simulink model "AFC_FFNN_trainlm_15_15_15_NoSat_Jan_23_RepFast"  (R2021a)
settings: Solver=ode15s  StartTime=0.0  StopTime=T  MaxStep=.01  RelTol=1e-3
undefined symbols (not defined in the file): AF_sensor_tol, fault_time, fuel_inj_tol, kappa_tol, MAF_sensor_tol, patch_sig, pump_tol, safe_patch_sig, sw, tau_ww_tol
libraries: neural x50, simulink x3
(part 2 of 2)

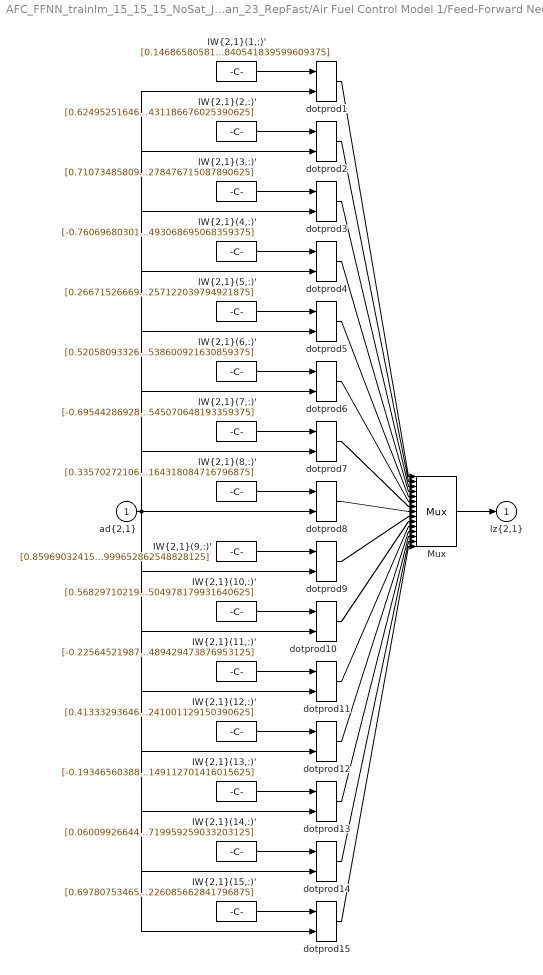
== system AFC_FFNN_trainlm_15_15_15_NoSat_Jan_23_RepFast/Air Fuel Control Model 1/Feed-Forward Neural Network/Layer 2/LW{2,1} ==
  "ad{2,1}" : Inport  PortDimensions=15
      mask Display: e = 0.06;c1 = [120 230 180]/255;c2 = ([120 230 180]+0)/(256+128);c3 = ([120 230 180]+128)/(256+128);patch([0 1 1 0],[0 0 1 1],c1);patch([0 1 1 1-e 1-e 0+e],[0 0 1 1-e 0+e 0+e],c2);patch([0 0 1 1-e 0+e 0+e],[0 1 1 1-e 1-e 0+e],c3);plot([0 1 1 0 0],[0 0 1 1 0]);
  "IW{2,1}(1,:)'" : Constant  Value=[0.1468658058110374753368887468241155147552490234375;-0.79986890826566170442646352967130951583385467529296875;-0.31412633700742986775367171503603458404541015625;-0.00332579596645567361623552216087773558683693408966064453125;0.1312237814313217398876076913438737392425537109375;0.344524720263148787058327116028522141277790069580078125;-0.0408263490105180704148324366542510688304901123046875;-0.197143189425145581861187338290619663894176483154296875;-0.211467920088183103377588167859357781708240509033203125;-0.0228887593846358594618095594341866672039031982421875;0.9727483047205953692326829695957712829113006591796875;-0.15275385755570081158793982467614114284515380859375;0.448998803742126473270701580986496992409229278564453125;0.1435643437851705783714351127855479717254638671875;0.9935339892538654904541317591792903840541839599609375]
      mask Display: e = 0.06;c1 = [120 150 230]/255;c2 = ([120 150 230]+0)/383;c3 = ([120 150 230]+128)/383;patch([0 1 1 0],[0 0 1 1],c1);patch([0 1 1 1-e 1-e 0+e],[0 0 1 1-e 0+e 0+e],c2);patch([0 0 1 1-e 0+e 0+e],[0 1 1 1-e 1-e 0+e],c3);plot([0 1 1 0 0],[0 0 1 1 0]);disp('weights');
  "IW{2,1}(10,:)'" : Constant  Value=[0.5682971021935003808067676800419576466083526611328125;-0.7275100622197581134997790286433883011341094970703125;1.4406360212981699220335940481163561344146728515625;-0.7098343326217027016156180252437479794025421142578125;0.3745290668992009575077872796100564301013946533203125;-0.0614067373898913027030488365198834799230098724365234375;0.964924509608335423394009922049008309841156005859375;-1.3273865141156055980076189371175132691860198974609375;-0.203156115681673465900303199305199086666107177734375;-0.7408998901019552274505031164153479039669036865234375;1.0233270938010277095742139863432385027408599853515625;0.69404582667213154945073938506538979709148406982421875;-0.23685294970424097815708819325664080679416656494140625;-0.0126849048783663764794482631259597837924957275390625;-0.244330775780726927592922947951592504978179931640625]
      mask Display: e = 0.06;c1 = [120 150 230]/255;c2 = ([120 150 230]+0)/383;c3 = ([120 150 230]+128)/383;patch([0 1 1 0],[0 0 1 1],c1);patch([0 1 1 1-e 1-e 0+e],[0 0 1 1-e 0+e 0+e],c2);patch([0 0 1 1-e 0+e 0+e],[0 1 1 1-e 1-e 0+e],c3);plot([0 1 1 0 0],[0 0 1 1 0]);disp('weights');
  "IW{2,1}(11,:)'" : Constant  Value=[-0.2256452198759715255249602705589495599269866943359375;0.727956654138967262923642920213751494884490966796875;-0.5453793247586904424650811051833443343639373779296875;0.547967139390781898811155770090408623218536376953125;-0.1828759723086506028266740031540393829345703125;0.9374135951140996070307664922438561916351318359375;0.87270401334910641111264339997433125972747802734375;0.853037029850580719170238808146677911281585693359375;0.1825800053059129790522518987927469424903392791748046875;-0.7678337019231407101216291266609914600849151611328125;0.421204976982361978254942869170918129384517669677734375;-0.0579419915609621638541426591473282314836978912353515625;0.5795506990507470757023611440672539174556732177734375;-0.477128967133783277176917181350290775299072265625;-0.670782654299447944623580042389221489429473876953125]
      mask Display: e = 0.06;c1 = [120 150 230]/255;c2 = ([120 150 230]+0)/383;c3 = ([120 150 230]+128)/383;patch([0 1 1 0],[0 0 1 1],c1);patch([0 1 1 1-e 1-e 0+e],[0 0 1 1-e 0+e 0+e],c2);patch([0 0 1 1-e 0+e 0+e],[0 1 1 1-e 1-e 0+e],c3);plot([0 1 1 0 0],[0 0 1 1 0]);disp('weights');
  "IW{2,1}(12,:)'" : Constant  Value=[0.41333293646864799342210972099564969539642333984375;-0.8616022116206336622923345203162170946598052978515625;-0.348616050190197535041392029597773216664791107177734375;-0.5692780055831174745861744668218307197093963623046875;0.9529144783762959480810650347848422825336456298828125;-1.0241829268729427671047460535191930830478668212890625;0.5831636473464032466296202983357943594455718994140625;0.499306613814386957006519196511362679302692413330078125;0.6451270201528844783211980029591359198093414306640625;0.2605675373402061012484409729950129985809326171875;-0.01491909072521746537631770479492843151092529296875;-0.167342895014342241122307086698128841817378997802734375;-0.562609182407641572609691138495691120624542236328125;-0.2562071576988582677358863293193280696868896484375;-0.3877593402600434391302997028105892241001129150390625]
      mask Display: e = 0.06;c1 = [120 150 230]/255;c2 = ([120 150 230]+0)/383;c3 = ([120 150 230]+128)/383;patch([0 1 1 0],[0 0 1 1],c1);patch([0 1 1 1-e 1-e 0+e],[0 0 1 1-e 0+e 0+e],c2);patch([0 0 1 1-e 0+e 0+e],[0 1 1 1-e 1-e 0+e],c3);plot([0 1 1 0 0],[0 0 1 1 0]);disp('weights');
  "IW{2,1}(13,:)'" : Constant  Value=[-0.1934656038895019580792222768650390207767486572265625;-0.2390404906948966068380713068108889274299144744873046875;-0.1199124406723394986595820910224574618041515350341796875;0.263449521186924773274995459360070526599884033203125;0.4440977442440028344350366751314140856266021728515625;0.53872301524054255761342346886522136628627777099609375;-0.2115765017478363763103743622195906937122344970703125;-0.6234500873564188250242068534134887158870697021484375;-0.35608968297847898298869040445424616336822509765625;-0.49677879715403161497988548944704234600067138671875;0.419241740090347481118016048640129156410694122314453125;-0.33564242304183000698003525030799210071563720703125;0.433229749317704027067321703725610859692096710205078125;0.460056404944834351766758118174038827419281005859375;-0.256260589179901021594787380308844149112701416015625]
      mask Display: e = 0.06;c1 = [120 150 230]/255;c2 = ([120 150 230]+0)/383;c3 = ([120 150 230]+128)/383;patch([0 1 1 0],[0 0 1 1],c1);patch([0 1 1 1-e 1-e 0+e],[0 0 1 1-e 0+e 0+e],c2);patch([0 0 1 1-e 0+e 0+e],[0 1 1 1-e 1-e 0+e],c3);plot([0 1 1 0 0],[0 0 1 1 0]);disp('weights');
  "IW{2,1}(14,:)'" : Constant  Value=[0.0600992664475967774961873146821744740009307861328125;-0.65050183753509538409076640164130367338657379150390625;1.362085994538364541739383639651350677013397216796875;0.042474272203300279804327743704561726190149784088134765625;-0.2568578517627091439834430275368504226207733154296875;0.81744135101609993743210225147777236998081207275390625;-0.2498833666170330314315606301533989608287811279296875;-0.10525015327370969286935320496922940947115421295166015625;0.03216246871763693560009045313563547097146511077880859375;-0.502647721643322942242093631648458540439605712890625;-0.3867159297211497648305567054194398224353790283203125;0.73794130222845388811236944093252532184123992919921875;0.023130893299841949473094615541413077153265476226806640625;0.1348448958576984324508885038085281848907470703125;-0.3121945271696671131422817779821343719959259033203125]
      mask Display: e = 0.06;c1 = [120 150 230]/255;c2 = ([120 150 230]+0)/383;c3 = ([120 150 230]+128)/383;patch([0 1 1 0],[0 0 1 1],c1);patch([0 1 1 1-e 1-e 0+e],[0 0 1 1-e 0+e 0+e],c2);patch([0 0 1 1-e 0+e 0+e],[0 1 1 1-e 1-e 0+e],c3);plot([0 1 1 0 0],[0 0 1 1 0]);disp('weights');
  "IW{2,1}(15,:)'" : Constant  Value=[0.6978075346578351823012553722946904599666595458984375;-0.73662106818013228792807467470993287861347198486328125;-1.1123650153279764918323735400917939841747283935546875;-0.11030835599876363806171042369896895252168178558349609375;0.734200051032391609595606496441178023815155029296875;-0.1876468311379226872048775476287119090557098388671875;0.7184828013258843792954166929121129214763641357421875;0.60013058592138601721188706505927257239818572998046875;0.053448907742239711027298909584715147502720355987548828125;0.9120261675330609829615013950387947261333465576171875;0.74302316527727463313368616582010872662067413330078125;-0.4149924922329122356501329704769887030124664306640625;0.8172177093320953655819494088063947856426239013671875;0.9305593583416114089601478553959168493747711181640625;-0.06823078255388548285509386914782226085662841796875]
      mask Display: e = 0.06;c1 = [120 150 230]/255;c2 = ([120 150 230]+0)/383;c3 = ([120 150 230]+128)/383;patch([0 1 1 0],[0 0 1 1],c1);patch([0 1 1 1-e 1-e 0+e],[0 0 1 1-e 0+e 0+e],c2);patch([0 0 1 1-e 0+e 0+e],[0 1 1 1-e 1-e 0+e],c3);plot([0 1 1 0 0],[0 0 1 1 0]);disp('weights');
  "IW{2,1}(2,:)'" : Constant  Value=[0.6249525164608675797950354535714723169803619384765625;0.412890681297754802425714615310425870120525360107421875;-0.2159788554806470750602187536060228012502193450927734375;0.3508923949942845954552694820449687540531158447265625;-0.1422183036643251963226930456585250794887542724609375;0.612312898614546075037878836155869066715240478515625;-0.48507316554088220073026604950428009033203125;-0.64878999441310247764391760938451625406742095947265625;-0.7391660575102572128258771044784225523471832275390625;-0.086116803229575378253457529353909194469451904296875;0.5698654964419118673646380557329393923282623291015625;0.7165517327928829782734965192503295838832855224609375;-0.464988407736367237443886324399500153958797454833984375;-0.6335294236047517291154917984385974705219268798828125;-0.0748668890844010892493542996817268431186676025390625]
      mask Display: e = 0.06;c1 = [120 150 230]/255;c2 = ([120 150 230]+0)/383;c3 = ([120 150 230]+128)/383;patch([0 1 1 0],[0 0 1 1],c1);patch([0 1 1 1-e 1-e 0+e],[0 0 1 1-e 0+e 0+e],c2);patch([0 0 1 1-e 0+e 0+e],[0 1 1 1-e 1-e 0+e],c3);plot([0 1 1 0 0],[0 0 1 1 0]);disp('weights');
  "IW{2,1}(3,:)'" : Constant  Value=[0.7107348580942822735551089863292872905731201171875;-0.342239153986161337428484330303035676479339599609375;-0.19023870928318320494554427568800747394561767578125;-0.8599175367517801760186557658016681671142578125;0.32990234960410713682676941971294581890106201171875;0.000120624052140971826929671806283295154571533203125;-0.5464970238293351822989052379853092133998870849609375;0.4014662532458366239751512694056145846843719482421875;0.2334039403776750898344971574260853230953216552734375;0.039564090317298905574716627597808837890625;-0.425583977343654940028727651224471628665924072265625;0.79559741585239596162182351690717041492462158203125;-0.183333770828677966591158110531978309154510498046875;-0.665380052920768516599991926341317594051361083984375;-0.09104362918916653057976873242296278476715087890625]
      mask Display: e = 0.06;c1 = [120 150 230]/255;c2 = ([120 150 230]+0)/383;c3 = ([120 150 230]+128)/383;patch([0 1 1 0],[0 0 1 1],c1);patch([0 1 1 1-e 1-e 0+e],[0 0 1 1-e 0+e 0+e],c2);patch([0 0 1 1-e 0+e 0+e],[0 1 1 1-e 1-e 0+e],c3);plot([0 1 1 0 0],[0 0 1 1 0]);disp('weights');
  "IW{2,1}(4,:)'" : Constant  Value=[-0.7606968030107481570922800528933294117450714111328125;-0.7535509674089102549743302006390877068042755126953125;-0.0455651968607446722359100022003985941410064697265625;-0.4725010400413507394290490992716513574123382568359375;0.7174803353217551471487922754022292792797088623046875;-0.3329299845408628666376671390025876462459564208984375;0.6842857552629875161898098667734302580356597900390625;-0.4818920562347488445453791428008116781711578369140625;0.8353636929366297092514059841050766408443450927734375;0.3770512178109644008117129487800411880016326904296875;0.7827280064979384999190870075835846364498138427734375;0.6009678795926596261978147595073096454143524169921875;-0.226909272979972431727446746663190424442291259765625;0.4638849660490063087081580306403338909149169921875;-0.6100135079769015700179579653195105493068695068359375]
      mask Display: e = 0.06;c1 = [120 150 230]/255;c2 = ([120 150 230]+0)/383;c3 = ([120 150 230]+128)/383;patch([0 1 1 0],[0 0 1 1],c1);patch([0 1 1 1-e 1-e 0+e],[0 0 1 1-e 0+e 0+e],c2);patch([0 0 1 1-e 0+e 0+e],[0 1 1 1-e 1-e 0+e],c3);plot([0 1 1 0 0],[0 0 1 1 0]);disp('weights');
  "IW{2,1}(5,:)'" : Constant  Value=[0.266715266696730513018565034144558012485504150390625;-0.332533963167412849326609602940152399241924285888671875;0.46985499617614345790883589870645664632320404052734375;-0.76651164888252265594559275996289215981960296630859375;-0.027119185528958755782014122814871370792388916015625;0.70201174892076012579167354488163255155086517333984375;-0.4255423106365061602929245054838247597217559814453125;-0.2801603963093963756136872689239680767059326171875;-1.091708492451566758774106347118504345417022705078125;-0.0635774578716965521607562550343573093414306640625;0.02153832134551721122495138160957139916718006134033203125;-0.5143365196906428682410705732763744890689849853515625;-0.67841812849830451792598751126206479966640472412109375;0.931788859196381213934046172653324902057647705078125;-0.0385504692749076838254040922038257122039794921875]
      mask Display: e = 0.06;c1 = [120 150 230]/255;c2 = ([120 150 230]+0)/383;c3 = ([120 150 230]+128)/383;patch([0 1 1 0],[0 0 1 1],c1);patch([0 1 1 1-e 1-e 0+e],[0 0 1 1-e 0+e 0+e],c2);patch([0 0 1 1-e 0+e 0+e],[0 1 1 1-e 1-e 0+e],c3);plot([0 1 1 0 0],[0 0 1 1 0]);disp('weights');
  "IW{2,1}(6,:)'" : Constant  Value=[0.5205809332657251875531301266164518892765045166015625;0.369459481161023450823677194421179592609405517578125;0.6135047231561936431631920640938915312290191650390625;0.059136244425769035615303437225520610809326171875;0.374148337822167054156352605787105858325958251953125;-0.9186599140957822928754694657982327044010162353515625;-0.599107887517563053592084543197415769100189208984375;-0.4882174416335660627197512440034188330173492431640625;-0.85474982889113704231931478716433048248291015625;-0.599702408658733698842979720211587846279144287109375;0.2338031628062349209784542836132459342479705810546875;0.4616289121641188319955517727066762745380401611328125;-0.3749002843746840341054848977364599704742431640625;-0.4338786459236596559918552884482778608798980712890625;0.885425136431036374773384522995911538600921630859375]
      mask Display: e = 0.06;c1 = [120 150 230]/255;c2 = ([120 150 230]+0)/383;c3 = ([120 150 230]+128)/383;patch([0 1 1 0],[0 0 1 1],c1);patch([0 1 1 1-e 1-e 0+e],[0 0 1 1-e 0+e 0+e],c2);patch([0 0 1 1-e 0+e 0+e],[0 1 1 1-e 1-e 0+e],c3);plot([0 1 1 0 0],[0 0 1 1 0]);disp('weights');
  "IW{2,1}(7,:)'" : Constant  Value=[-0.695442869286326814659560113796032965183258056640625;-0.881550976945969733122865363839082419872283935546875;0.8093922409587241961759218611405231058597564697265625;0.09552673732521850535892582456654054112732410430908203125;0.4068000332342711633515364155755378305912017822265625;0.37250243473358002344042461118078790605068206787109375;0.6941789590380762486887533668777905404567718505859375;0.63902927140569254493840389841352589428424835205078125;-0.396592890196696412630217309924773871898651123046875;-0.5169744106628451074669783338322304189205169677734375;-0.60043822969177307324883940964355133473873138427734375;0.55133135124757604028644664140301756560802459716796875;0.1855228100993589201994637960524414665997028350830078125;-0.7646540500302252407749392659752629697322845458984375;-0.5250407508751633312016338095418177545070648193359375]
      mask Display: e = 0.06;c1 = [120 150 230]/255;c2 = ([120 150 230]+0)/383;c3 = ([120 150 230]+128)/383;patch([0 1 1 0],[0 0 1 1],c1);patch([0 1 1 1-e 1-e 0+e],[0 0 1 1-e 0+e 0+e],c2);patch([0 0 1 1-e 0+e 0+e],[0 1 1 1-e 1-e 0+e],c3);plot([0 1 1 0 0],[0 0 1 1 0]);disp('weights');
  "IW{2,1}(8,:)'" : Constant  Value=[0.335702721066147180550842676893807947635650634765625;-0.6234135387209367440419782724347896873950958251953125;0.05600270005710324128234134377635200507938861846923828125;0.738664641377198449845309369266033172607421875;-0.8518457958148861752789571255561895668506622314453125;0.1699491832068246999210003878033603541553020477294921875;0.9024625642331134400819792062975466251373291015625;0.1858132442856689492405308783418149687349796295166015625;-0.83828507014463971014350818222737871110439300537109375;0.336524452681205676896070144721306860446929931640625;-0.62012758117489708009628657237044535577297210693359375;0.6610380858166651218965625957935117185115814208984375;-0.009806907065873525508603592015788308344781398773193359375;-0.012782031693472806210820635897107422351837158203125;0.2179003717440213261369308384018950164318084716796875]
      mask Display: e = 0.06;c1 = [120 150 230]/255;c2 = ([120 150 230]+0)/383;c3 = ([120 150 230]+128)/383;patch([0 1 1 0],[0 0 1 1],c1);patch([0 1 1 1-e 1-e 0+e],[0 0 1 1-e 0+e 0+e],c2);patch([0 0 1 1-e 0+e 0+e],[0 1 1 1-e 1-e 0+e],c3);plot([0 1 1 0 0],[0 0 1 1 0]);disp('weights');
  "IW{2,1}(9,:)'" : Constant  Value=[0.8596903241516711258185523547581396996974945068359375;0.5446400156727084773677916018641553819179534912109375;-8.868221093991540016077124164439737796783447265625;-0.63033703012778452556830188768799416720867156982421875;0.2101733469269653209465786858345381915569305419921875;0.6476803619839068826280481516732834279537200927734375;-0.884327548513141881159071999718435108661651611328125;0.45028320308204128341600380736053921282291412353515625;-0.61726588006551230680685193874523974955081939697265625;0.8963735042713738554454039331176318228244781494140625;-0.66039547280161359221750672077178023755550384521484375;-0.1518690387460164270549967113765887916088104248046875;-0.0875557235233536956808819695652346126735210418701171875;-0.32870025966817717488765993039123713970184326171875;-0.7543531819149951189729108591563999652862548828125]
      mask Display: e = 0.06;c1 = [120 150 230]/255;c2 = ([120 150 230]+0)/383;c3 = ([120 150 230]+128)/383;patch([0 1 1 0],[0 0 1 1],c1);patch([0 1 1 1-e 1-e 0+e],[0 0 1 1-e 0+e 0+e],c2);patch([0 0 1 1-e 0+e 0+e],[0 1 1 1-e 1-e 0+e],c3);plot([0 1 1 0 0],[0 0 1 1 0]);disp('weights');
  Mux : Mux  Inputs=15
      mask Display: e = 0.06;c1 = [120 150 230]/255;c2 = ([120 150 230]+0)/383;c3 = ([120 150 230]+128)/383;patch([0 1 1 0],[0 0 1 1],c1);patch([0 1 1 1-e 1-e 0+e],[0 0 1 1-e 0+e 0+e],c2);patch([0 0 1 1-e 0+e 0+e],[0 1 1 1-e 1-e 0+e],c3);plot([0 1 1 0 0],[0 0 1 1 0]);disp('Mux');
  dotprod{1..15} (15 alike) : neural/Weight Functions/dotprod
  "lz{2,1}" : Outport
      mask Display: e = 0.06;c1 = [120 230 180]/255;c2 = ([120 230 180]+0)/(256+128);c3 = ([120 230 180]+128)/(256+128);patch([0 1 1 0],[0 0 1 1],c1);patch([0 1 1 1-e 1-e 0+e],[0 0 1 1-e 0+e 0+e],c2);patch([0 0 1 1-e 0+e 0+e],[0 1 1 1-e 1-e 0+e],c3);plot([0 1 1 0 0],[0 0 1 1 0]);
  wires:
  "IW{2,1}(1,:)'"/1 -> dotprod1/1
  "ad{2,1}"/1 -> dotprod1/2, dotprod2/2, dotprod3/2, dotprod4/2, dotprod5/2, dotprod6/2, dotprod7/2, dotprod8/2, dotprod9/2, dotprod10/2, dotprod11/2, dotprod12/2, dotprod13/2, dotprod14/2, dotprod15/2
  dotprod1/1 -> Mux/1
  "IW{2,1}(2,:)'"/1 -> dotprod2/1
  dotprod2/1 -> Mux/2
  "IW{2,1}(3,:)'"/1 -> dotprod3/1
  dotprod3/1 -> Mux/3
  "IW{2,1}(4,:)'"/1 -> dotprod4/1
  dotprod4/1 -> Mux/4
  "IW{2,1}(5,:)'"/1 -> dotprod5/1
  dotprod5/1 -> Mux/5
  "IW{2,1}(6,:)'"/1 -> dotprod6/1
  dotprod6/1 -> Mux/6
  "IW{2,1}(7,:)'"/1 -> dotprod7/1
  dotprod7/1 -> Mux/7
  "IW{2,1}(8,:)'"/1 -> dotprod8/1
  dotprod8/1 -> Mux/8
  "IW{2,1}(9,:)'"/1 -> dotprod9/1
  dotprod9/1 -> Mux/9
  "IW{2,1}(10,:)'"/1 -> dotprod10/1
  dotprod10/1 -> Mux/10
  "IW{2,1}(11,:)'"/1 -> dotprod11/1
  dotprod11/1 -> Mux/11
  "IW{2,1}(12,:)'"/1 -> dotprod12/1
  dotprod12/1 -> Mux/12
  "IW{2,1}(13,:)'"/1 -> dotprod13/1
  dotprod13/1 -> Mux/13
  "IW{2,1}(14,:)'"/1 -> dotprod14/1
  dotprod14/1 -> Mux/14
  "IW{2,1}(15,:)'"/1 -> dotprod15/1
  dotprod15/1 -> Mux/15
  Mux/1 -> "lz{2,1}"/1

== system AFC_FFNN_trainlm_15_15_15_NoSat_Jan_23_RepFast/Air Fuel Control Model 1/Feed-Forward Neural Network/Layer 3/Delays 1 ==
  "p{3}" : Inport  PortDimensions=15
      mask Display: e = 0.06;c1 = [120 230 180]/255;c2 = ([120 230 180]+0)/(256+128);c3 = ([120 230 180]+128)/(256+128);patch([0 1 1 0],[0 0 1 1],c1);patch([0 1 1 1-e 1-e 0+e],[0 0 1 1-e 0+e 0+e],c2);patch([0 0 1 1-e 0+e 0+e],[0 1 1 1-e 1-e 0+e],c3);plot([0 1 1 0 0],[0 0 1 1 0]);
  mux : Mux  Inputs=1
      mask Display: e = 0.06;c1 = [120 150 230]/255;c2 = ([120 150 230]+0)/383;c3 = ([120 150 230]+128)/383;patch([0 1 1 0],[0 0 1 1],c1);patch([0 1 1 1-e 1-e 0+e],[0 0 1 1-e 0+e 0+e],c2);patch([0 0 1 1-e 0+e 0+e],[0 1 1 1-e 1-e 0+e],c3);plot([0 1 1 0 0],[0 0 1 1 0]);disp('Mux')
  "pd{3,2}" : Outport
      mask Display: e = 0.06;c1 = [120 230 180]/255;c2 = ([120 230 180]+0)/(256+128);c3 = ([120 230 180]+128)/(256+128);patch([0 1 1 0],[0 0 1 1],c1);patch([0 1 1 1-e 1-e 0+e],[0 0 1 1-e 0+e 0+e],c2);patch([0 0 1 1-e 0+e 0+e],[0 1 1 1-e 1-e 0+e],c3);plot([0 1 1 0 0],[0 0 1 1 0]);
  wires:
  "p{3}"/1 -> mux/1
  mux/1 -> "pd{3,2}"/1

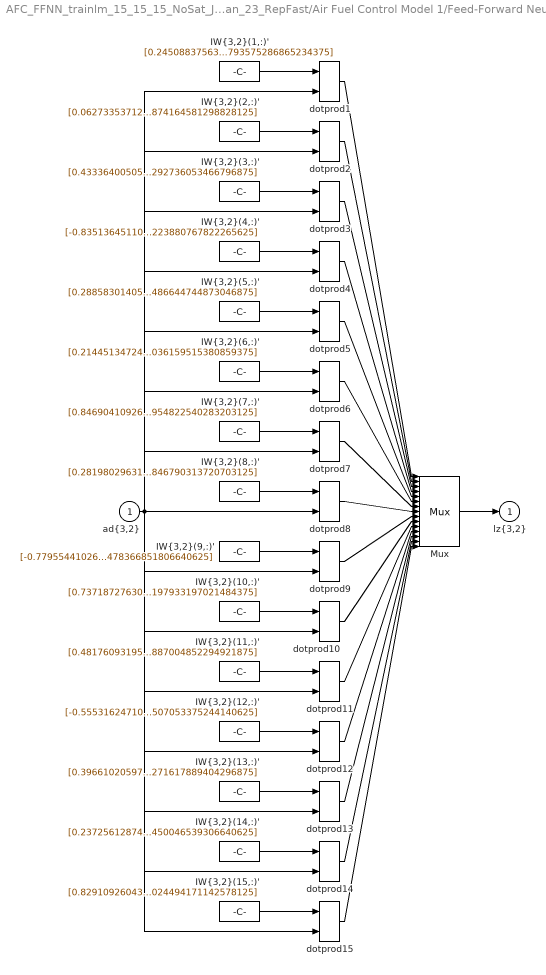
== system AFC_FFNN_trainlm_15_15_15_NoSat_Jan_23_RepFast/Air Fuel Control Model 1/Feed-Forward Neural Network/Layer 3/LW{3,2} ==
  "ad{3,2}" : Inport  PortDimensions=15
      mask Display: e = 0.06;c1 = [120 230 180]/255;c2 = ([120 230 180]+0)/(256+128);c3 = ([120 230 180]+128)/(256+128);patch([0 1 1 0],[0 0 1 1],c1);patch([0 1 1 1-e 1-e 0+e],[0 0 1 1-e 0+e 0+e],c2);patch([0 0 1 1-e 0+e 0+e],[0 1 1 1-e 1-e 0+e],c3);plot([0 1 1 0 0],[0 0 1 1 0]);
  "IW{3,2}(1,:)'" : Constant  Value=[0.245088375632908306300805634236894547939300537109375;-0.9630654315301534484916601286386139690876007080078125;0.9600091175752567540513382482458837330341339111328125;0.845118910397417710811396318604238331317901611328125;-0.7176582003307065971142719718045555055141448974609375;-0.589273318857662875558389714569784700870513916015625;-0.953421768699953542380853832582943141460418701171875;0.1957236320591506650856672422378323972225189208984375;0.1829565434390272304909785816562362015247344970703125;-0.7818743407298061054433446770417504012584686279296875;-0.93223551791788850096054375171661376953125;0.426672705339178559569290882791392505168914794921875;0.662323204252165620431469506002031266689300537109375;-0.25531274000819781377913386677391827106475830078125;0.3872106486699615768287685568793676793575286865234375]
      mask Display: e = 0.06;c1 = [120 150 230]/255;c2 = ([120 150 230]+0)/383;c3 = ([120 150 230]+128)/383;patch([0 1 1 0],[0 0 1 1],c1);patch([0 1 1 1-e 1-e 0+e],[0 0 1 1-e 0+e 0+e],c2);patch([0 0 1 1-e 0+e 0+e],[0 1 1 1-e 1-e 0+e],c3);plot([0 1 1 0 0],[0 0 1 1 0]);disp('weights');
  "IW{3,2}(10,:)'" : Constant  Value=[0.73718727630584368615274115654756315052509307861328125;-0.2004073980385996656128355652981554158031940460205078125;0.8725744369771657460432834341190755367279052734375;0.2950234375494618088708875802694819867610931396484375;0.70820415272860881561456380950403399765491485595703125;-0.8684387029046580774860331075615249574184417724609375;-0.15133362262805427622680554122780449688434600830078125;0.5128555425635241693527177631040103733539581298828125;0.147533983117959233144489417099975980818271636962890625;-0.273037612577155475168666498575475998222827911376953125;0.11870394445328828758601247272963519208133220672607421875;-0.8691350869650136257149597440729849040508270263671875;0.61262970314491360657171981074498035013675689697265625;0.50163527702638333050089158859918825328350067138671875;-0.59102917099452001448156579499482177197933197021484375]
      mask Display: e = 0.06;c1 = [120 150 230]/255;c2 = ([120 150 230]+0)/383;c3 = ([120 150 230]+128)/383;patch([0 1 1 0],[0 0 1 1],c1);patch([0 1 1 1-e 1-e 0+e],[0 0 1 1-e 0+e 0+e],c2);patch([0 0 1 1-e 0+e 0+e],[0 1 1 1-e 1-e 0+e],c3);plot([0 1 1 0 0],[0 0 1 1 0]);disp('weights');
  "IW{3,2}(11,:)'" : Constant  Value=[0.481760931953577442587999257739284075796604156494140625;0.1308495322055307219510922323024715296924114227294921875;0.9318956526707997678471429026103578507900238037109375;0.4618391492819784449608278009691275656223297119140625;-0.77317191553957897998117232418735511600971221923828125;-0.7025786881286404383928356764954514801502227783203125;0.036866405706285819421363925130208372138440608978271484375;-0.691165200016234937407944016740657389163970947265625;0.34409448820270238655893990653567016124725341796875;-0.337813293653005775052378112377482466399669647216796875;0.36330954121183989258270230493508279323577880859375;-0.744147449247748227207921445369720458984375;0.303146505633484775188435378368012607097625732421875;-0.336689663055434740268623272640979848802089691162109375;-0.187992897187381657886362518183887004852294921875]
      mask Display: e = 0.06;c1 = [120 150 230]/255;c2 = ([120 150 230]+0)/383;c3 = ([120 150 230]+128)/383;patch([0 1 1 0],[0 0 1 1],c1);patch([0 1 1 1-e 1-e 0+e],[0 0 1 1-e 0+e 0+e],c2);patch([0 0 1 1-e 0+e 0+e],[0 1 1 1-e 1-e 0+e],c3);plot([0 1 1 0 0],[0 0 1 1 0]);disp('weights');
  "IW{3,2}(12,:)'" : Constant  Value=[-0.55531624710789440069191869042697362601757049560546875;-0.84963676770620744083117870104615576565265655517578125;0.2268727209830530000544968061149120330810546875;-0.8786502692251316748439649018109776079654693603515625;0.476458690685954866506079952159780077636241912841796875;0.702457526197160841974209688487462699413299560546875;-0.74048004099400899225003058745642192661762237548828125;-0.21594212458759753925363611415377818048000335693359375;0.44632579800651839274650001243571750819683074951171875;0.7383300189650441325284191407263278961181640625;0.8820809561430558165540105619584210216999053955078125;-0.009417987396717342196694744416163302958011627197265625;0.9593706355644731065268615566310472786426544189453125;0.021950583480834839900097676945733837783336639404296875;0.98673458107807976436021135668852366507053375244140625]
      mask Display: e = 0.06;c1 = [120 150 230]/255;c2 = ([120 150 230]+0)/383;c3 = ([120 150 230]+128)/383;patch([0 1 1 0],[0 0 1 1],c1);patch([0 1 1 1-e 1-e 0+e],[0 0 1 1-e 0+e 0+e],c2);patch([0 0 1 1-e 0+e 0+e],[0 1 1 1-e 1-e 0+e],c3);plot([0 1 1 0 0],[0 0 1 1 0]);disp('weights');
  "IW{3,2}(13,:)'" : Constant  Value=[0.396610205975270968536960936035029590129852294921875;0.4450747945940218830429557783645577728748321533203125;-0.9064537320609000747850814150297082960605621337890625;-0.163812813249240907254034027573652565479278564453125;-0.3703825082072469410121584587614051997661590576171875;0.8023027323506948249587367172352969646453857421875;0.26350475742635826037485458073206245899200439453125;0.544613936845101509476307910517789423465728759765625;0.401119941632610110815448933863081037998199462890625;0.5401045509741078110010903401416726410388946533203125;-0.8917352280379529094744839312625117599964141845703125;0.3017691597321772167816789078642614185810089111328125;-0.4867945875125208043954216918791644275188446044921875;-0.6526665617479745495899123852723278105258941650390625;0.6857794558071137469568157030153088271617889404296875]
      mask Display: e = 0.06;c1 = [120 150 230]/255;c2 = ([120 150 230]+0)/383;c3 = ([120 150 230]+128)/383;patch([0 1 1 0],[0 0 1 1],c1);patch([0 1 1 1-e 1-e 0+e],[0 0 1 1-e 0+e 0+e],c2);patch([0 0 1 1-e 0+e 0+e],[0 1 1 1-e 1-e 0+e],c3);plot([0 1 1 0 0],[0 0 1 1 0]);disp('weights');
  "IW{3,2}(14,:)'" : Constant  Value=[0.237256128742527661046324283233843743801116943359375;0.9380274187991322065727217704989016056060791015625;0.0866903145212971626420994653017260134220123291015625;0.0578359415262996723328114967443980276584625244140625;0.9294309917431651246744195304927416145801544189453125;-0.8816609086055173793994299558107741177082061767578125;-0.4715985768164510094635488712810911238193511962890625;-0.460748141201527072752242020214907824993133544921875;-0.41891407817934211976762526319362223148345947265625;-0.3783130093030127039099852481740526854991912841796875;-0.8492849071904544633326850089360959827899932861328125;-0.0794995693271440817539996714913286268711090087890625;-0.3383663648992041306229339170386083424091339111328125;-0.43337226352280300289976366912014782428741455078125;-0.948715584742816364638429149636067450046539306640625]
      mask Display: e = 0.06;c1 = [120 150 230]/255;c2 = ([120 150 230]+0)/383;c3 = ([120 150 230]+128)/383;patch([0 1 1 0],[0 0 1 1],c1);patch([0 1 1 1-e 1-e 0+e],[0 0 1 1-e 0+e 0+e],c2);patch([0 0 1 1-e 0+e 0+e],[0 1 1 1-e 1-e 0+e],c3);plot([0 1 1 0 0],[0 0 1 1 0]);disp('weights');
  "IW{3,2}(15,:)'" : Constant  Value=[0.82910926043546118169302872047410346567630767822265625;0.71055847709559050162653193183359690010547637939453125;0.9487008142226667217755675665102899074554443359375;0.474919090886384065441916391137056052684783935546875;-0.0710109317395639372261229027571971528232097625732421875;-0.19957001056105472258650479489006102085113525390625;-0.51220007739129835844238414210849441587924957275390625;0.8029325061854368783542668097652494907379150390625;0.951399203755272093729900007019750773906707763671875;-0.51364246249228207030768089680350385606288909912109375;0.202332976998175817495706496629281900823116302490234375;-0.59847790243299225920736716943792998790740966796875;0.67639255299290612644114162321784533560276031494140625;0.96738750446996080167849640929489396512508392333984375;0.63976603321324809758863239039783366024494171142578125]
      mask Display: e = 0.06;c1 = [120 150 230]/255;c2 = ([120 150 230]+0)/383;c3 = ([120 150 230]+128)/383;patch([0 1 1 0],[0 0 1 1],c1);patch([0 1 1 1-e 1-e 0+e],[0 0 1 1-e 0+e 0+e],c2);patch([0 0 1 1-e 0+e 0+e],[0 1 1 1-e 1-e 0+e],c3);plot([0 1 1 0 0],[0 0 1 1 0]);disp('weights');
  "IW{3,2}(2,:)'" : Constant  Value=[0.06273353712899344680753443981302552856504917144775390625;0.21838741136412431753655027932836674153804779052734375;0.8207439236663989223785620197304524481296539306640625;-0.736546191755028445413699955679476261138916015625;0.425698497602584657872881734874681569635868072509765625;0.8786358923690469335809893891564570367336273193359375;-0.901476841034734466262534624547697603702545166015625;-0.46577999141781345482371534671983681619167327880859375;-0.76229697559826992137033130347845144569873809814453125;-0.50212144541077641246573648459161631762981414794921875;-0.85377769073226283946809189728810451924800872802734375;-0.217996527540531948030633202506578527390956878662109375;-0.9290875196453820539232992814504541456699371337890625;0.470420996218344711348180453569511882960796356201171875;0.29250657955589887126990333854337222874164581298828125]
      mask Display: e = 0.06;c1 = [120 150 230]/255;c2 = ([120 150 230]+0)/383;c3 = ([120 150 230]+128)/383;patch([0 1 1 0],[0 0 1 1],c1);patch([0 1 1 1-e 1-e 0+e],[0 0 1 1-e 0+e 0+e],c2);patch([0 0 1 1-e 0+e 0+e],[0 1 1 1-e 1-e 0+e],c3);plot([0 1 1 0 0],[0 0 1 1 0]);disp('weights');
  "IW{3,2}(3,:)'" : Constant  Value=[0.433364005051513512256633475772105157375335693359375;0.91843299975869097107050720296683721244335174560546875;-0.6131501670085708344259955993038602173328399658203125;0.888148439859744343038983060978353023529052734375;1.0113064787332870508862470160238444805145263671875;-0.747263229640165338452106880140490829944610595703125;0.3861434377850232468887270442792214453220367431640625;-0.95418754909423764143383550617727451026439666748046875;-0.012624631593664260853504544002134934999048709869384765625;0.2119925710532757079374022168849478475749492645263671875;-0.1767059813408740354123693805377115495502948760986328125;-0.52772463648005896175163798034191131591796875;0.1226645475719867206532143200092832557857036590576171875;-0.031984137788055234941086979461033479310572147369384765625;0.09553484489950007929603970069365459494292736053466796875]
      mask Display: e = 0.06;c1 = [120 150 230]/255;c2 = ([120 150 230]+0)/383;c3 = ([120 150 230]+128)/383;patch([0 1 1 0],[0 0 1 1],c1);patch([0 1 1 1-e 1-e 0+e],[0 0 1 1-e 0+e 0+e],c2);patch([0 0 1 1-e 0+e 0+e],[0 1 1 1-e 1-e 0+e],c3);plot([0 1 1 0 0],[0 0 1 1 0]);disp('weights');
  "IW{3,2}(4,:)'" : Constant  Value=[-0.8351364511086585284971306464285589754581451416015625;0.1621631799288543174242249733651988208293914794921875;0.5409734433553128329918990857549943029880523681640625;0.2721665852208321467742280219681560993194580078125;-0.771798802527578597931778858765028417110443115234375;-0.070369737464647474922685432829894125461578369140625;-0.1597043763150962636387930615455843508243560791015625;0.8153583337968919320104532744153402745723724365234375;-0.0956253000795233010222773373243398964405059814453125;-0.0823858345236889721974193889764137566089630126953125;-0.063419533625113100328007931238971650600433349609375;0.6024625168200776759164227769360877573490142822265625;0.748422067764029197434183515724726021289825439453125;-0.9169422073506112713658922075410373508930206298828125;0.4545960387774954369888291694223880767822265625]
      mask Display: e = 0.06;c1 = [120 150 230]/255;c2 = ([120 150 230]+0)/383;c3 = ([120 150 230]+128)/383;patch([0 1 1 0],[0 0 1 1],c1);patch([0 1 1 1-e 1-e 0+e],[0 0 1 1-e 0+e 0+e],c2);patch([0 0 1 1-e 0+e 0+e],[0 1 1 1-e 1-e 0+e],c3);plot([0 1 1 0 0],[0 0 1 1 0]);disp('weights');
  "IW{3,2}(5,:)'" : Constant  Value=[0.288583014054416386873214150909916497766971588134765625;-0.5823159927174847982911387589410878717899322509765625;-0.1205428831065702421909691111068241298198699951171875;0.5718050437108728178969840882928110659122467041015625;-0.05707982322478259706866055012142169289290904998779296875;0.0234614928237093511853572636027820408344268798828125;0.72468308084190702356153224172885529696941375732421875;-0.65592120331648928743817350550671108067035675048828125;0.66407056206940062725863072046195156872272491455078125;0.237296575775909623917669932779972441494464874267578125;-0.07350729081963496003293556668722885660827159881591796875;-0.5155593734253012261348203537636436522006988525390625;0.68344748498616192389221168923540972173213958740234375;-1.065036341660235308381743379868566989898681640625;-0.5708474801027019207566581826540641486644744873046875]
      mask Display: e = 0.06;c1 = [120 150 230]/255;c2 = ([120 150 230]+0)/383;c3 = ([120 150 230]+128)/383;patch([0 1 1 0],[0 0 1 1],c1);patch([0 1 1 1-e 1-e 0+e],[0 0 1 1-e 0+e 0+e],c2);patch([0 0 1 1-e 0+e 0+e],[0 1 1 1-e 1-e 0+e],c3);plot([0 1 1 0 0],[0 0 1 1 0]);disp('weights');
  "IW{3,2}(6,:)'" : Constant  Value=[0.21445134724792414004923557513393461704254150390625;0.899792657956907770966381576727144420146942138671875;-0.281123313723487200377348926849663257598876953125;0.1741749122148050776814898199518211185932159423828125;-0.5183807483678410932270708144642412662506103515625;0.6288552804994032019436644986853934824466705322265625;0.465227198924214768727125601799343712627887725830078125;-0.0588479104270755726258101958592305891215801239013671875;0.6924687200416539401004456522059626877307891845703125;0.094545475218808461281838617651374079287052154541015625;0.51500092154636245567189689609222114086151123046875;0.044553065233051414306686410782276652753353118896484375;-0.3291801677997601149883166726795025169849395751953125;-0.2377577604319738302507403204799629747867584228515625;0.124791079182933584146297789629898034036159515380859375]
      mask Display: e = 0.06;c1 = [120 150 230]/255;c2 = ([120 150 230]+0)/383;c3 = ([120 150 230]+128)/383;patch([0 1 1 0],[0 0 1 1],c1);patch([0 1 1 1-e 1-e 0+e],[0 0 1 1-e 0+e 0+e],c2);patch([0 0 1 1-e 0+e 0+e],[0 1 1 1-e 1-e 0+e],c3);plot([0 1 1 0 0],[0 0 1 1 0]);disp('weights');
  "IW{3,2}(7,:)'" : Constant  Value=[0.84690410926559411830538692811387591063976287841796875;-0.57644694882305314020953801446012221276760101318359375;0.592245801338891819654008941142819821834564208984375;-0.218728148045378656405546280439011752605438232421875;0.3998644107718869467049671584391035139560699462890625;0.0408120069936763751883290751720778644084930419921875;0.364846337384792718250281495784292928874492645263671875;0.78113830619367252694473791052587330341339111328125;0.7134007305407958909881926956586539745330810546875;-0.49645646502253859555509052370325662195682525634765625;-0.11134820182172307234669261788440053351223468780517578125;0.424094819243451881529693991979002021253108978271484375;0.52870836873802862232452071111765690147876739501953125;0.92199124713394831065471635156427510082721710205078125;0.278029218606783257161652045397204346954822540283203125]
      mask Display: e = 0.06;c1 = [120 150 230]/255;c2 = ([120 150 230]+0)/383;c3 = ([120 150 230]+128)/383;patch([0 1 1 0],[0 0 1 1],c1);patch([0 1 1 1-e 1-e 0+e],[0 0 1 1-e 0+e 0+e],c2);patch([0 0 1 1-e 0+e 0+e],[0 1 1 1-e 1-e 0+e],c3);plot([0 1 1 0 0],[0 0 1 1 0]);disp('weights');
  "IW{3,2}(8,:)'" : Constant  Value=[0.281980296311453992874618279529386200010776519775390625;-0.49098615925635635814927582032396458089351654052734375;0.1501377451791918726797803174122236669063568115234375;-0.43846370282760727121740274014882743358612060546875;-0.3760599355484668393501124228350818157196044921875;0.7102539399932836783335687869112007319927215576171875;0.64505924706654471645350668040919117629528045654296875;0.6807406223311842641265911879600025713443756103515625;0.917404760094499227562891974230296909809112548828125;-0.75727524876828355981928098117350600659847259521484375;-0.471479998670810085403815037352615036070346832275390625;0.7698899977264199723236970385187305510044097900390625;0.3561512930510704055819815039285458624362945556640625;0.478612215957272046917836405555135570466518402099609375;0.66607923937361956934211093539488501846790313720703125]
      mask Display: e = 0.06;c1 = [120 150 230]/255;c2 = ([120 150 230]+0)/383;c3 = ([120 150 230]+128)/383;patch([0 1 1 0],[0 0 1 1],c1);patch([0 1 1 1-e 1-e 0+e],[0 0 1 1-e 0+e 0+e],c2);patch([0 0 1 1-e 0+e 0+e],[0 1 1 1-e 1-e 0+e],c3);plot([0 1 1 0 0],[0 0 1 1 0]);disp('weights');
  "IW{3,2}(9,:)'" : Constant  Value=[-0.7795544102685294518551017972640693187713623046875;-0.30086235279490181060424447423429228365421295166015625;0.9389629483296195733288413975969888269901275634765625;0.4652989588579530266798656157334335148334503173828125;0.71002720009645858834090859090792946517467498779296875;0.19849170235196567091406905092298984527587890625;0.09045032559771927493930121499943197704851627349853515625;0.06670678777794532277045647106206160970032215118408203125;-0.58470791868755134235158266164944507181644439697265625;-0.34975348577461440324753993991180323064327239990234375;-0.6911154251049593799649528591544367372989654541015625;0.0337011677262120112885668277158401906490325927734375;0.56950625081418804196431437958381138741970062255859375;0.802397984495051286302214066381566226482391357421875;0.351001708368221587708291053786524571478366851806640625]
      mask Display: e = 0.06;c1 = [120 150 230]/255;c2 = ([120 150 230]+0)/383;c3 = ([120 150 230]+128)/383;patch([0 1 1 0],[0 0 1 1],c1);patch([0 1 1 1-e 1-e 0+e],[0 0 1 1-e 0+e 0+e],c2);patch([0 0 1 1-e 0+e 0+e],[0 1 1 1-e 1-e 0+e],c3);plot([0 1 1 0 0],[0 0 1 1 0]);disp('weights');
  Mux : Mux  Inputs=15
      mask Display: e = 0.06;c1 = [120 150 230]/255;c2 = ([120 150 230]+0)/383;c3 = ([120 150 230]+128)/383;patch([0 1 1 0],[0 0 1 1],c1);patch([0 1 1 1-e 1-e 0+e],[0 0 1 1-e 0+e 0+e],c2);patch([0 0 1 1-e 0+e 0+e],[0 1 1 1-e 1-e 0+e],c3);plot([0 1 1 0 0],[0 0 1 1 0]);disp('Mux');
  dotprod{1..15} (15 alike) : neural/Weight Functions/dotprod
  "lz{3,2}" : Outport
      mask Display: e = 0.06;c1 = [120 230 180]/255;c2 = ([120 230 180]+0)/(256+128);c3 = ([120 230 180]+128)/(256+128);patch([0 1 1 0],[0 0 1 1],c1);patch([0 1 1 1-e 1-e 0+e],[0 0 1 1-e 0+e 0+e],c2);patch([0 0 1 1-e 0+e 0+e],[0 1 1 1-e 1-e 0+e],c3);plot([0 1 1 0 0],[0 0 1 1 0]);
  wires:
  "IW{3,2}(1,:)'"/1 -> dotprod1/1
  "ad{3,2}"/1 -> dotprod1/2, dotprod2/2, dotprod3/2, dotprod4/2, dotprod5/2, dotprod6/2, dotprod7/2, dotprod8/2, dotprod9/2, dotprod10/2, dotprod11/2, dotprod12/2, dotprod13/2, dotprod14/2, dotprod15/2
  dotprod1/1 -> Mux/1
  "IW{3,2}(2,:)'"/1 -> dotprod2/1
  dotprod2/1 -> Mux/2
  "IW{3,2}(3,:)'"/1 -> dotprod3/1
  dotprod3/1 -> Mux/3
  "IW{3,2}(4,:)'"/1 -> dotprod4/1
  dotprod4/1 -> Mux/4
  "IW{3,2}(5,:)'"/1 -> dotprod5/1
  dotprod5/1 -> Mux/5
  "IW{3,2}(6,:)'"/1 -> dotprod6/1
  dotprod6/1 -> Mux/6
  "IW{3,2}(7,:)'"/1 -> dotprod7/1
  dotprod7/1 -> Mux/7
  "IW{3,2}(8,:)'"/1 -> dotprod8/1
  dotprod8/1 -> Mux/8
  "IW{3,2}(9,:)'"/1 -> dotprod9/1
  dotprod9/1 -> Mux/9
  "IW{3,2}(10,:)'"/1 -> dotprod10/1
  dotprod10/1 -> Mux/10
  "IW{3,2}(11,:)'"/1 -> dotprod11/1
  dotprod11/1 -> Mux/11
  "IW{3,2}(12,:)'"/1 -> dotprod12/1
  dotprod12/1 -> Mux/12
  "IW{3,2}(13,:)'"/1 -> dotprod13/1
  dotprod13/1 -> Mux/13
  "IW{3,2}(14,:)'"/1 -> dotprod14/1
  dotprod14/1 -> Mux/14
  "IW{3,2}(15,:)'"/1 -> dotprod15/1
  dotprod15/1 -> Mux/15
  Mux/1 -> "lz{3,2}"/1

== system AFC_FFNN_trainlm_15_15_15_NoSat_Jan_23_RepFast/Air Fuel Control Model 1/Feed-Forward Neural Network/Layer 4/Delays 1 ==
  "p{4}" : Inport  PortDimensions=15
      mask Display: e = 0.06;c1 = [120 230 180]/255;c2 = ([120 230 180]+0)/(256+128);c3 = ([120 230 180]+128)/(256+128);patch([0 1 1 0],[0 0 1 1],c1);patch([0 1 1 1-e 1-e 0+e],[0 0 1 1-e 0+e 0+e],c2);patch([0 0 1 1-e 0+e 0+e],[0 1 1 1-e 1-e 0+e],c3);plot([0 1 1 0 0],[0 0 1 1 0]);
  mux : Mux  Inputs=1
      mask Display: e = 0.06;c1 = [120 150 230]/255;c2 = ([120 150 230]+0)/383;c3 = ([120 150 230]+128)/383;patch([0 1 1 0],[0 0 1 1],c1);patch([0 1 1 1-e 1-e 0+e],[0 0 1 1-e 0+e 0+e],c2);patch([0 0 1 1-e 0+e 0+e],[0 1 1 1-e 1-e 0+e],c3);plot([0 1 1 0 0],[0 0 1 1 0]);disp('Mux')
  "pd{4,3}" : Outport
      mask Display: e = 0.06;c1 = [120 230 180]/255;c2 = ([120 230 180]+0)/(256+128);c3 = ([120 230 180]+128)/(256+128);patch([0 1 1 0],[0 0 1 1],c1);patch([0 1 1 1-e 1-e 0+e],[0 0 1 1-e 0+e 0+e],c2);patch([0 0 1 1-e 0+e 0+e],[0 1 1 1-e 1-e 0+e],c3);plot([0 1 1 0 0],[0 0 1 1 0]);
  wires:
  "p{4}"/1 -> mux/1
  mux/1 -> "pd{4,3}"/1

== system AFC_FFNN_trainlm_15_15_15_NoSat_Jan_23_RepFast/Air Fuel Control Model 1/Feed-Forward Neural Network/Layer 4/LW{4,3} ==
  "ad{4,3}" : Inport  PortDimensions=15
      mask Display: e = 0.06;c1 = [120 230 180]/255;c2 = ([120 230 180]+0)/(256+128);c3 = ([120 230 180]+128)/(256+128);patch([0 1 1 0],[0 0 1 1],c1);patch([0 1 1 1-e 1-e 0+e],[0 0 1 1-e 0+e 0+e],c2);patch([0 0 1 1-e 0+e 0+e],[0 1 1 1-e 1-e 0+e],c3);plot([0 1 1 0 0],[0 0 1 1 0]);
  "IW{4,3}(1,:)'" : Constant  Value=[0.2591334396422422248207340089720673859119415283203125;0.012145859162768744832217038265298469923436641693115234375;0.1685450539412977899456080876916530542075634002685546875;-0.2765298080445297568275009325589053332805633544921875;-0.036949552461770042433020222460982040502130985260009765625;0.7348019150720601633253181717009283602237701416015625;0.66752533765158406087181219845660962164402008056640625;-0.506805264805141320039183483459055423736572265625;-0.774119525201343972042877794592641294002532958984375;0.57916351889194606084032557191676460206508636474609375;0.47108707011460138058822622042498551309108734130859375;0.206935503787299357458806525755790062248706817626953125;0.9049118192961653761585694155655801296234130859375;-0.5921463917838043489183519341167993843555450439453125;-0.89208973526663026820671120731276459991931915283203125]
      mask Display: e = 0.06;c1 = [120 150 230]/255;c2 = ([120 150 230]+0)/383;c3 = ([120 150 230]+128)/383;patch([0 1 1 0],[0 0 1 1],c1);patch([0 1 1 1-e 1-e 0+e],[0 0 1 1-e 0+e 0+e],c2);patch([0 0 1 1-e 0+e 0+e],[0 1 1 1-e 1-e 0+e],c3);plot([0 1 1 0 0],[0 0 1 1 0]);disp('weights');
  Mux : Mux  Inputs=1
      mask Display: e = 0.06;c1 = [120 150 230]/255;c2 = ([120 150 230]+0)/383;c3 = ([120 150 230]+128)/383;patch([0 1 1 0],[0 0 1 1],c1);patch([0 1 1 1-e 1-e 0+e],[0 0 1 1-e 0+e 0+e],c2);patch([0 0 1 1-e 0+e 0+e],[0 1 1 1-e 1-e 0+e],c3);plot([0 1 1 0 0],[0 0 1 1 0]);disp('Mux');
  dotprod1 : neural/Weight Functions/dotprod
  "lz{4,3}" : Outport
      mask Display: e = 0.06;c1 = [120 230 180]/255;c2 = ([120 230 180]+0)/(256+128);c3 = ([120 230 180]+128)/(256+128);patch([0 1 1 0],[0 0 1 1],c1);patch([0 1 1 1-e 1-e 0+e],[0 0 1 1-e 0+e 0+e],c2);patch([0 0 1 1-e 0+e 0+e],[0 1 1 1-e 1-e 0+e],c3);plot([0 1 1 0 0],[0 0 1 1 0]);
  wires:
  "IW{4,3}(1,:)'"/1 -> dotprod1/1
  "ad{4,3}"/1 -> dotprod1/2
  dotprod1/1 -> Mux/1
  Mux/1 -> "lz{4,3}"/1
